simulink model "PMSM_FOC"  (R2022b)
settings: Solver=VariableStepAuto  StartTime=0.0  StopTime=10  MaxStep=1e-6  RelTol=1e-3
values from neighbouring files (symbols this model uses):
  Bm = 0    [PMSM_FOC_parameters.m]
  downlimit_iq = -Vdc/sqrt(3)    [PMSM_FOC_parameters.m]
  downlimit_w = -1.2*Tn    (= -0.357696)    [PMSM_FOC_parameters.m]
  dt = Ts    (= 5e-05)    [PMSM_FOC_parameters.m]
  F = 0.0001    [PMSM_FOC_parameters.m]
  fwb = 50    [PMSM_FOC_parameters.m]
  In = 9.2    [PMSM_FOC_parameters.m]
  J = 0.21e-4    (= 2.1e-05)    [PMSM_FOC_parameters.m]
  ki_iq = Rs*wc    (= 879.645943005)    [PMSM_FOC_parameters.m]
  ki_w = kp_w*wsc/5    (= 1.33977738742)    [PMSM_FOC_parameters.m]
  kp_iq = Lq*wc    (= 0.753982236862)    [PMSM_FOC_parameters.m]
  kp_w = J*wsc/K    (= 0.0213232193851)    [PMSM_FOC_parameters.m]
  ks_iq = 1.5*kp_iq    (= 1.13097335529)    [PMSM_FOC_parameters.m]
  ks_w = 1.5*kp_w    (= 0.0319848290776)    [PMSM_FOC_parameters.m]
  Ld = 0.12e-3    (= 0.00012)    [PMSM_FOC_parameters.m]
  Lq = 0.12e-3    (= 0.00012)    [PMSM_FOC_parameters.m]
  Ls = Ld    (= 0.00012)    [PMSM_FOC_parameters.m]
  n = 3000    [PMSM_FOC_parameters.m]
  p = 4    [PMSM_FOC_parameters.m]
  phis = 0.0054    [PMSM_FOC_parameters.m]
  Rs = 0.14    [PMSM_FOC_parameters.m]
  Tn = 1.5*p*phis*In    (= 0.29808)    [PMSM_FOC_parameters.m]
  Ts = 1/fc    (= 5e-05)    [PMSM_FOC_parameters.m]
  uplimit_iq = Vdc/sqrt(3)    [PMSM_FOC_parameters.m]
  uplimit_w = 1.2*Tn    (= 0.357696)    [PMSM_FOC_parameters.m]
  Vdc = 24    [PMSM_FOC_parameters.m]
undefined symbols (not defined in the file or in its folder): DiscIntNeverNeededParam
libraries: dspsrcs4 x2, spsACVoltageSourceLib x1, spsAlphaBetaZerotodq0Lib x1, simulink x1, spsDCVoltageSourceLib x1, spsPermanentMagnetSynchronousMachineLib x1, spsThreePhaseVIMeasurementLib x1, spsUniversalBridgeLib x1, spsVoltageMeasurementLib x1, spsabctoAlphaBetaZeroLib x1, spsdq0toAlphaBetaZeroLib x1, spspowerguiLib x1
settings Model: Creator=OptiPlex 7090  LastModifiedBy=OptiPlex 7090
settings DebuggingCC: AlgebraicLoopMsg=none  UnconnectedInputMsg=warning  UnconnectedOutputMsg=warning  UnconnectedLineMsg=warning  SFMachineParentedDataDiag=warning
settings ModelReferenceCC: EnableRefExpFcnMdlSchedulingChecks=on
settings RTWCC: DLArmComputeVersion=19.05

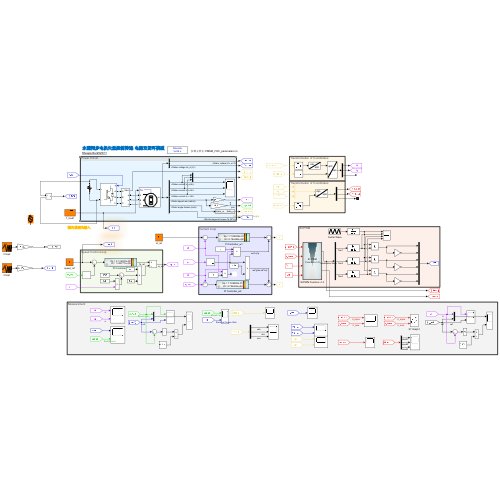
[thumbnail: Simulink's stored preview of the top-level diagram]
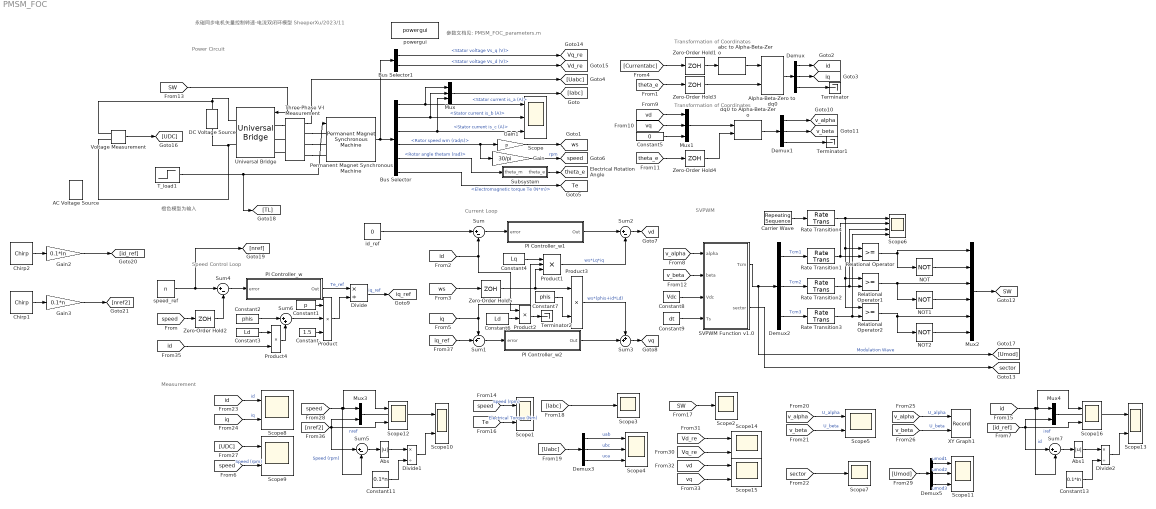
== system PMSM_FOC ==
  note: 参数文档见: PMSM_FOC_parameters.m
  note: Measurement
  note: SVPWM
  note: Speed Control Loop
  note: 橙色模型为输入
  note: Current Loop
  note: Transformation of Coordinates
  note: Power Circuit
  note: 永磁同步电机矢量控制转速-电流双闭环模型
      | SheeperXu/2023/11
  note: Transformation of Coordinates
  AC Voltage Source : spsACVoltageSourceLib/AC Voltage Source  Amplitude=Vdc*0.1  Phase=0  Frequency=500  SampleTime=0  Measurements=None  BusType=swing  Pref=10e3  Qref=0  Qmin=-inf  Qmax=+inf
  Abs : Abs  SaturateOnIntegerOverflow=off
  Abs1 : Abs  SaturateOnIntegerOverflow=off
  Alpha-Beta-Zero to dq0 : spsAlphaBetaZerotodq0Lib/Alpha-Beta-Zero to dq0  Alignment=Aligned with phase A axis
  Bus Selector : BusSelector  OutputSignals=Stator current is_a (A),Stator current is_b (A),Stator current is_c (A),Rotor speed wm (rad/s),Rotor angle thetam (rad),Electromagnetic torque Te (N*m)
  Bus Selector1 : BusSelector  OutputSignals=Stator voltage Vs_q (V),Stator voltage Vs_d (V)
  Carrier Wave : simulink/Sources/Repeating Sequence  rep_seq_t=[0 Ts/2 Ts]  rep_seq_y=[0 Ts/2 0]
  Chirp1 : dspsrcs4/Chirp  sweep=Linear  mode=Unidirectional  f0=0  f1=500  t1=10  Tsweep=10  phase=0  Ts=dt  spf=1  datatype=Double  OutputFrames=off
  Chirp2 : dspsrcs4/Chirp  sweep=Linear  mode=Unidirectional  f0=0  f1=5000  t1=10  Tsweep=10  phase=0  Ts=dt  spf=1  datatype=Double  OutputFrames=off
  Constant : Constant  Value=1.5
  Constant1 : Constant  Value=p
  Constant11 : Constant  Value=0.1*n
  Constant13 : Constant  Value=0.1*In
  Constant2 : Constant  Value=phis
  Constant3 : Constant  Value=Ld
  Constant4 : Constant  Value=Lq
  Constant5 : Constant  Value=0
  Constant6 : Constant  Value=Ld
  Constant7 : Constant  Value=phis
  Constant8 : Constant  Value=Vdc
  Constant9 : Constant  Value=dt
  DC Voltage Source : spsDCVoltageSourceLib/DC Voltage Source  Amplitude=Vdc  Measurements=None
  Demux{,1..3,5} (5 alike) : Demux  Outputs=3
  Divide : Product  Inputs=*/
  Divide1 : Product  Inputs=*/
  Divide2 : Product  Inputs=*/
  Gain : Gain  Gain=30/pi
  Gain1 : Gain  Gain=p
  Gain2 : Gain  Gain=0.1*In
  Gain3 : Gain  Gain=0.1*n
  Mux : Mux  Inputs=3
  Mux1 : Mux  Inputs=3
  Mux2 : Mux  Inputs=6
  Mux3 : Mux  Inputs=2
  Mux4 : Mux  Inputs=2
  NOT : Logic  Operator=NOT  IconShape=distinctive  AllPortsSameDT=off  OutDataTypeStr=boolean
  NOT1 : Logic  Operator=NOT  IconShape=distinctive  AllPortsSameDT=off  OutDataTypeStr=boolean
  NOT2 : Logic  Operator=NOT  IconShape=distinctive  AllPortsSameDT=off  OutDataTypeStr=boolean
  PI Controller_w : Subsystem  mask{Kp=kp_w, Ki=ki_w, Ks=ks_w, uplimit=uplimit_w, downlimit=downlimit_w, SampleTime=1/fwb}
      mask prompts: uplimit "Up_Limit"; downlimit "Down_Limit"; SampleTime "Sample_Time(s)"
      mask DialogControl DescTextVar Prompt: PI Controller
      mask DialogControl ParameterGroupVar Prompt: 参数
      mask DialogControl Control2 Prompt: PI Controller Parameters
      mask Display:
      | image('PI.png');
      | fprintf('Kp = %d\n Ki= %d', Kp, Ki);
  PI Controller_w1 : Subsystem  mask{Kp=kp_iq, Ki=ki_iq, Ks=ks_iq, uplimit=uplimit_iq, downlimit=downlimit_iq, SampleTime=dt}
      mask prompts: uplimit "Up_Limit"; downlimit "Down_Limit"; SampleTime "Sample_Time(s)"
      mask DialogControl DescTextVar Prompt: PI Controller
      mask DialogControl ParameterGroupVar Prompt: 参数
      mask DialogControl Control2 Prompt: PI Controller Parameters
      mask Display:
      | image('PI.png');
      | fprintf('Kp = %d\n Ki= %d', Kp, Ki);
  PI Controller_w2 : Subsystem  mask{Kp=kp_iq, Ki=ki_iq, Ks=ks_iq, uplimit=uplimit_iq, downlimit=downlimit_iq, SampleTime=dt}
      mask prompts: uplimit "Up_Limit"; downlimit "Down_Limit"; SampleTime "Sample_Time(s)"
      mask DialogControl DescTextVar Prompt: PI Controller
      mask DialogControl ParameterGroupVar Prompt: 参数
      mask DialogControl Control2 Prompt: PI Controller Parameters
      mask Display:
      | image('PI.png');
      | fprintf('Kp = %d\n Ki= %d', Kp, Ki);
  Permanent Magnet Synchronous Machine : spsPermanentMagnetSynchronousMachineLib/Permanent Magnet Synchronous Machine  NbPhases=3  FluxDistribution=Sinusoidal  RotorType=Salient-pole  MechanicalLoad=Torque Tm  PresetModel=No  ShowDetailedParameters=on  MeasurementBus=off  Resistance=Rs  Inductance=8.5e-3  dqInductances=[Ld,Lq]  La=[Ls]  MachineConstant=Flux linkage established by magnets (V.s)  Flux=phis  VoltageCst=3.9178  TorqueCst=0.0324  Flat=120  Mechanical=[J F p 0]  PolePairs=4  InitialConditions=[0,0, 0,0]  InitialConditions5ph=[0 0 0 0 0 0]  RefAngle=Aligned with phase A axis (original Park)  IterativeDiscreteModel=Trapezoidal non iterative  TsBlock=-1  TsPowergui=0
  Product : Product  Inputs=3
  Product1 : Product  Inputs=3
  Product2 : Product
  Product3 : Product
  Product4 : Product
  Rate Transition{1..4} (4 alike) : RateTransition  Deterministic=off
  Relational Operator : RelationalOperator  OutDataTypeStr=boolean  RndMeth=Simplest  InputSameDT=off
  Relational Operator1 : RelationalOperator  OutDataTypeStr=boolean  RndMeth=Simplest  InputSameDT=off
  Relational Operator2 : RelationalOperator  OutDataTypeStr=boolean  RndMeth=Simplest  InputSameDT=off
  SVPWM Function v1.0 : MATLAB Function  TreatAsAtomicUnit=on
  Scope : Scope  NumInputPorts=3
  Scope{1,5,8..10,12..16} (10 alike) : Scope  NumInputPorts=2
  Scope11 : Scope  NumInputPorts=3
  Scope2 : Scope
  Scope3 : Scope
  Scope4 : Scope  NumInputPorts=3
  Scope6 : Scope  NumInputPorts=4
  Scope7 : Scope
  Subsystem : Subsystem
  Sum{,2,4..5,7} (5 alike) : Sum  Inputs=|+-
  Sum1 : Sum  Inputs=-+|
  Sum3 : Sum  Inputs=++|
  Sum6 : Sum  Inputs=|++
  T_load1 : Step  Time=0  Before=0.3*Tn  After=0.3*Tn  SampleTime=dt
  Terminator : Terminator
  Terminator1 : Terminator
  Terminator2 : Terminator
  Three-Phase V-I Measurement : spsThreePhaseVIMeasurementLib/Three-Phase V-I Measurement  VoltageMeasurement=phase-to-phase  SetLabelV=off  LabelV=Vabc  Vpu=off  VpuLL=off  CurrentMeasurement=yes  SetLabelI=on  LabelI=Currentabc  Ipu=off  Pbase=100e6  Vbase=500e3  OutputType=Complex  PhasorSimulation=off  PSBequivalent=0
  Universal Bridge : spsUniversalBridgeLib/Universal Bridge  Arms=3  SnubberResistance=1e5  SnubberCapacitance=inf  Device=IGBT / Diodes  Ron=0.001  Lon=0  ForwardVoltages="[  0  0  ]"  ForwardVoltage=0  GTOparameters=[ 10e-6 , 20e-6 ]  IGBTparameters=[ 1e-6 , 2e-6 ]  Measurements=Device voltages  Measurements_2=None  converterType=Rectifier
  Voltage Measurement : spsVoltageMeasurementLib/Voltage Measurement  PhasorSimulation=off  OutputType=Complex  PSBequivalent=0
  XY Graph1 : Record  FileSettingsInternal="{\"entries\":[{\"content\":{\"excelSettings\":{\"content\":{},\"type\":\"Streamout.ExcelSettings\"}},\"type\":\"Streamout.FileSettingStorage\",\"uuid\":\"a06b98c5-8dbe-469b-b57c-4ceb2281ba3f\"}],\"packageUris\":[\"http://schema.mathworks.com/mf0/streamout_blocks/R2020a\"],\"version\":\"1.0\"}"  Layout=[1 1]  SignalsInternal="{\"entries\":[{\"content\":{\"signals\":[{\"content\":{\"blockPath\":[\"PMSM_FOC/XY Graph1\"],\"channel\":[],\"dimensions\":[1],\"domain\":\"PMSM_FOC/XY Graph1\",\"lineColor\":\"#a2142f\",\"plots\":[1],\"port\":1,\"sid\":[],\"signalID\":17,\"signalName\":\"U_alpha\"},\"type\":\"RecordBlkView.Signal\",\"uuid\":\"add1d3f9-caf3-41c6-8cfa-02cf336879b9\"},{\"content\":{\"blockPath\":[\"PMSM_FOC/XY Graph1\"],\"channel\":[],\"dimensions\":[1],\"domain\":\"PMSM_FOC/XY Graph1\",\"lineColor\":\"#139fff\",\"plots\":[1],\"port\":2,\"sid\":[],\"signalID\":20,\"signalName\":\"U_beta\"},\"type\":\"RecordBlkView.Signal\",\"uuid\":\"8e1dd278-356f-4010-8d5d-71b90ce6082a\"}]},\"type\":\"RecordBlkView.InputSignals\",\"uuid\":\"6cc1d440-9683-4637-b98a-52bf58c64516\"}],\"packageUris\":[\"http://schema.mathworks.com/mf0/streamout_blocks/R2020a\"],\"version\":\"1.0\"}"  VisualizationBindings="{\"xyplotplugin\":{\"info\":[{\"series\":[{\"bindingParametersList\":[{\"parameter\":\"X-Axis\",\"signalID\":17,\"signalName\":\"U_alpha\"},{\"parameter\":\"Y-Axis\",\"signalID\":20,\"signalName\":\"U_beta\"}],\"seriesID\":6900}],\"subplotID\":1}]}}"  CompatibilityTag=XY  st=-1
  Zero-Order Hold{1..5} (5 alike) : ZeroOrderHold  SampleTime=dt
  abc to Alpha-Beta-Zero : spsabctoAlphaBetaZeroLib/abc to Alpha-Beta-Zero
  dq0 to Alpha-Beta-Zero : spsdq0toAlphaBetaZeroLib/dq0 to Alpha-Beta-Zero  Alignment=Aligned with phase A axis
  id_ref : Constant  Value=0
  powergui : spspowerguiLib/powergui  Priority=1  SimulationMode=Discrete  SampleTime=1e-6  frequency=60  Iterations=50  frequencyindice=0  Pbase=100e6  ErrMax=1e-4  UnitsV=kV  UnitsW=MW  buscounter=0  FunctionMessages=off  echomessages=off  EnableUseOfTLC=off  CurrentSourceSwitches=off  DisableSnubberDevices=off  DisableRonSwitches=off  DisableVfSwitches=off  DisplayEquations=off  AutomaticDiscreteSolvers=off  SolverType=Tustin/Backward Euler (TBE)  Interpol=off  ExternalGateDelay=off  methode=off  Ts=100  x0status=blocks  SPID=on  SwTol=0  HookPort=off  NonlinearTolerance=1e-4  nMaxIteration=100  ContinueOnMaxIteration=off  RestoreLinks=warning  ResistiveCurrentMeasurement=off  Frange=[0:2:500]  Ylog=off  Xlog=on  ShowGrid=off  save=off  variable=ZData  structure=0  ZoomFFT=off  StartTime=0.0  cycles=1  DisplayStyle=1  fundamental=60  FreqAxis=off  MaxFrequency=1000  frequencyindicesteady=1  RmsSteady=1  display=off
  speed_ref : Constant  Value=n
  tag scope: SW=global, Te=global, Vd_re=global, Vq_re=global, id=global, iq=global, iq_ref=global, sector=global, speed=global, theta_e=global, v_alpha=global, v_beta=global, vd=global, vq=global, ws=global
  wires:
  Permanent Magnet Synchronous Machine/1 -> Bus Selector/1, Bus Selector1/1
  Bus Selector/2 -> Mux/2, Scope/2  "<Stator current is_b (A)>"
  Bus Selector/1 -> Scope/1, Mux/1  "<Stator current is_a (A)>"
  Bus Selector/3 -> Scope/3, Mux/3  "<Stator current is_c (A)>"
  Bus Selector/4 -> Gain/1, Gain1/1  "<Rotor speed wm (rad/s)>"
  Mux/1 -> [Iabc]
  [Currentabc] -> Zero-Order Hold1/1
  abc to Alpha-Beta-Zero/1 -> Alpha-Beta-Zero to dq0/1
  Alpha-Beta-Zero to dq0/1 -> Demux/1
  Demux/1 -> [id]
  Demux/2 -> [iq]
  Gain2/1 -> [id_ref]
  T_load1/1 -> [TL], Permanent Magnet Synchronous Machine/1
  Sum/1 -> PI Controller_w1/1(error)
  PI Controller_w1/1(Out) -> Sum2/1
  Sum1/1 -> PI Controller_w2/1(error)
  Sum4/1 -> PI Controller_w/1(error)
  Bus Selector/5 -> Subsystem/1(theta_m)  "<Rotor angle thetam (rad)>"
  [speed] -> Zero-Order Hold2/1
  Zero-Order Hold1/1 -> abc to Alpha-Beta-Zero/1
  [theta_e] -> Zero-Order Hold3/1
  Subsystem/1(theta_e) -> [theta_e]
  Gain/1 -> [speed]  "rpm"
  Bus Selector/6 -> [Te]  "<Electromagnetic torque Te (N*m)>"
  Zero-Order Hold2/1 -> Sum4/2
  Zero-Order Hold3/1 -> Alpha-Beta-Zero to dq0/2
  PI Controller_w/1(Out) -> Divide/1  "Te_ref"
  Constant1/1 -> Product/1
  Product/1 -> Divide/2
  Gain1/1 -> [ws]
  Constant4/1 -> Product1/1
  [ws] -> Zero-Order Hold5/1
  PI Controller_w2/1(Out) -> Sum3/2
  [iq] -> Product1/2, Sum1/1
  [id] -> Sum/2, Product2/1
  Constant6/1 -> Product2/2
  Zero-Order Hold5/1 -> Product3/1, Product1/3
  Product1/1 -> Sum2/2  "ws*Lq*iq"
  Product3/1 -> Sum3/1  "ws*(phis+id*Ld)"
  Constant2/1 -> Sum6/1
  Sum6/1 -> Product/2
  Constant3/1 -> Product4/1
  Product4/1 -> Sum6/2
  Constant/1 -> Product/3
  Sum2/1 -> [vd]
  Sum3/1 -> [vq]
  Divide/1 -> [iq_ref]  "iq_ref"
  Mux1/1 -> dq0 to Alpha-Beta-Zero/1
  [vd] -> Mux1/1
  [vq] -> Mux1/2
  Constant5/1 -> Mux1/3
  [theta_e] -> Zero-Order Hold4/1
  Zero-Order Hold4/1 -> dq0 to Alpha-Beta-Zero/2
  dq0 to Alpha-Beta-Zero/1 -> Demux1/1
  Demux1/1 -> [v_alpha]
  Demux1/2 -> [v_beta]
  [v_alpha] -> SVPWM Function v1.0/1(alpha)
  [v_beta] -> SVPWM Function v1.0/2(beta)
  [SW] -> Universal Bridge/1
  Constant8/1 -> SVPWM Function v1.0/3(Vdc)
  Constant9/1 -> SVPWM Function v1.0/4(Ts)
  [speed] -> Scope1/1  "Speed (rpm)"
  Demux/3 -> Terminator/1
  Demux1/3 -> Terminator1/1
  [SW] -> Scope2/1
  [Iabc] -> Scope3/1
  [v_alpha] -> Scope5/1  "U_alpha"
  [v_beta] -> Scope5/2  "U_beta"
  Demux2/1 -> Rate Transition1/1  "Tcm1"
  Demux2/2 -> Rate Transition2/1  "Tcm2"
  Demux2/3 -> Rate Transition3/1  "Tcm3"
  Relational Operator/1 -> Mux2/1, NOT/1
  Relational Operator1/1 -> NOT1/1, Mux2/3
  Relational Operator2/1 -> Mux2/5, NOT2/1
  Mux2/1 -> [SW]
  SVPWM Function v1.0/1(Tcm) -> Demux2/1, [Umod]  "Modulation Wave"
  SVPWM Function v1.0/2(sector) -> [sector]
  [sector] -> Scope7/1
  [id] -> Scope8/1  "id"
  [iq] -> Scope8/2  "iq"
  [Uabc] -> Demux3/1
  Demux3/1 -> Scope4/1  "uab"
  [v_alpha] -> XY Graph1/1  "U_alpha"
  [v_beta] -> XY Graph1/2  "U_beta"
  Demux3/2 -> Scope4/2  "ubc"
  Demux3/3 -> Scope4/3  "uca"
  Three-Phase V-I Measurement/1 -> [Uabc]
  Carrier Wave/1 -> Rate Transition4/1
  Rate Transition1/1 -> Scope6/2, Relational Operator/2
  Rate Transition2/1 -> Scope6/3, Relational Operator1/2
  Rate Transition3/1 -> Scope6/4, Relational Operator2/2
  [Umod] -> Demux5/1
  Demux5/2 -> Scope11/2  "umod2"
  Demux5/1 -> Scope11/1  "umod1"
  Demux5/3 -> Scope11/3  "umod3"
  Bus Selector1/1 -> [Vq_re]  "<Stator voltage Vs_q (V)>"
  Bus Selector1/2 -> [Vd_re]  "<Stator voltage Vs_d (V)>"
  [Vd_re] -> Scope14/1
  [Vq_re] -> Scope14/2
  [vd] -> Scope15/1
  [vq] -> Scope15/2
  [id] -> Product4/2
  Rate Transition4/1 -> Relational Operator2/1, Relational Operator1/1, Relational Operator/1, Scope6/1
  Constant7/1 -> Product3/2
  Product2/1 -> Terminator2/1
  Voltage Measurement/1 -> [UDC]
  [UDC] -> Scope9/1
  [speed] -> Scope9/2  "Speed (rpm)"
  [speed] -> Sum5/2, Scope12/1, Mux3/1  "Speed (rpm)"
  [nref2] -> Scope12/2, Mux3/2, Sum5/1  "nref"
  [Te] -> Scope1/2  "Electrical Torque (Nm)"
  speed_ref/1 -> [nref], Sum4/1
  Mux3/1 -> Scope10/1
  Sum5/1 -> Abs/1
  NOT/1 -> Mux2/2
  NOT1/1 -> Mux2/4
  NOT2/1 -> Mux2/6
  Abs/1 -> Divide1/1
  Constant11/1 -> Divide1/2
  Divide1/1 -> Scope10/2
  Chirp1/1 -> Gain3/1
  Abs1/1 -> Divide2/1
  Constant13/1 -> Divide2/2
  Divide2/1 -> Scope13/2
  [id_ref] -> Scope16/2, Mux4/2, Sum7/1  "iref"
  [id] -> Sum7/2, Scope16/1, Mux4/1  "id"
  Mux4/1 -> Scope13/1
  Sum7/1 -> Abs1/1
  Chirp2/1 -> Gain2/1
  id_ref/1 -> Sum/1
  [iq_ref] -> Sum1/2
  Gain3/1 -> [nref2]
  connections:
  DC Voltage Source/RConn1 -- Voltage Measurement/LConn1 -- Universal Bridge/RConn1
  Universal Bridge/LConn1 -- Three-Phase V-I Measurement/LConn1
  Three-Phase V-I Measurement/LConn2 -- Universal Bridge/LConn2
  Three-Phase V-I Measurement/LConn3 -- Universal Bridge/LConn3
  Three-Phase V-I Measurement/RConn1 -- Permanent Magnet Synchronous Machine/LConn1
  Three-Phase V-I Measurement/RConn2 -- Permanent Magnet Synchronous Machine/LConn2
  Three-Phase V-I Measurement/RConn3 -- Permanent Magnet Synchronous Machine/LConn3
  Voltage Measurement/LConn2 -- DC Voltage Source/LConn1 -- Universal Bridge/RConn2

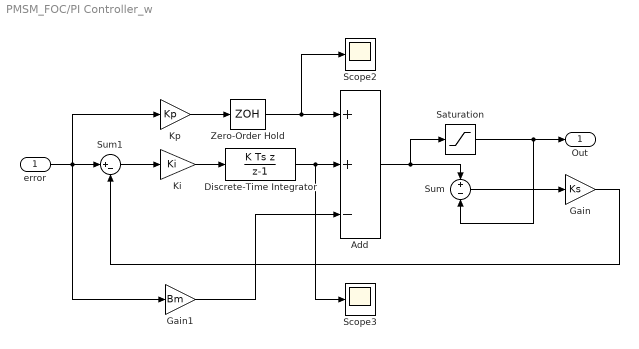
== system PMSM_FOC/PI Controller_w ==
  error : Inport
  Add : Sum  Inputs=++-
  Discrete-Time Integrator : DiscreteIntegrator  IntegratorMethod=Integration: Backward Euler  SampleTime=dt  LimitOutput=on  UpperSaturationLimit=uplimit  LowerSaturationLimit=downlimit  ICPrevOutput=DiscIntNeverNeededParam  ICPrevScaledInput=DiscIntNeverNeededParam
  Gain : Gain  Gain=Ks
  Gain1 : Gain  Gain=Bm
  Ki : Gain  Gain=Ki
  Kp : Gain  Gain=Kp
  Saturation : Saturate  UpperLimit=uplimit  LowerLimit=downlimit
  Scope2 : Scope
  Scope3 : Scope
  Sum : Sum  Inputs=+|-
  Sum1 : Sum  Inputs=|+-
  Zero-Order Hold : ZeroOrderHold  SampleTime=dt
  Out : Outport
  wires:
  Kp/1 -> Zero-Order Hold/1
  error/1 -> Gain1/1, Sum1/1, Kp/1
  Zero-Order Hold/1 -> Scope2/1, Add/1
  Add/1 -> Saturation/1, Sum/1
  Saturation/1 -> Sum/2, Out/1
  Sum/1 -> Gain/1
  Gain/1 -> Sum1/2
  Sum1/1 -> Ki/1
  Ki/1 -> Discrete-Time Integrator/1
  Discrete-Time Integrator/1 -> Scope3/1, Add/2
  Gain1/1 -> Add/3

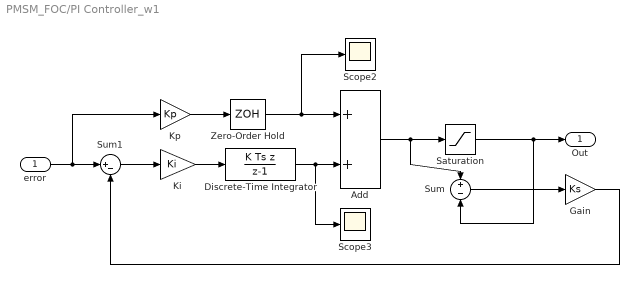
== system PMSM_FOC/PI Controller_w1 ==
  error : Inport
  Add : Sum
  Discrete-Time Integrator : DiscreteIntegrator  IntegratorMethod=Integration: Backward Euler  SampleTime=dt  LimitOutput=on  UpperSaturationLimit=uplimit  LowerSaturationLimit=downlimit  ICPrevOutput=DiscIntNeverNeededParam  ICPrevScaledInput=DiscIntNeverNeededParam
  Gain : Gain  Gain=Ks
  Ki : Gain  Gain=Ki
  Kp : Gain  Gain=Kp
  Saturation : Saturate  UpperLimit=uplimit  LowerLimit=downlimit
  Scope2 : Scope
  Scope3 : Scope
  Sum : Sum  Inputs=+|-
  Sum1 : Sum  Inputs=|+-
  Zero-Order Hold : ZeroOrderHold  SampleTime=dt
  Out : Outport
  wires:
  Discrete-Time Integrator/1 -> Add/2, Scope3/1
  Ki/1 -> Discrete-Time Integrator/1
  Sum1/1 -> Ki/1
  Gain/1 -> Sum1/2
  Sum/1 -> Gain/1
  Saturation/1 -> Out/1, Sum/2
  Add/1 -> Saturation/1, Sum/1
  Zero-Order Hold/1 -> Scope2/1, Add/1
  error/1 -> Kp/1, Sum1/1
  Kp/1 -> Zero-Order Hold/1

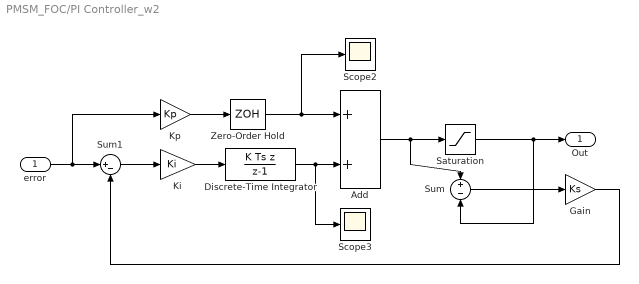
== system PMSM_FOC/PI Controller_w2 ==
  error : Inport
  Add : Sum
  Discrete-Time Integrator : DiscreteIntegrator  IntegratorMethod=Integration: Backward Euler  SampleTime=dt  LimitOutput=on  UpperSaturationLimit=uplimit  LowerSaturationLimit=downlimit  ICPrevOutput=DiscIntNeverNeededParam  ICPrevScaledInput=DiscIntNeverNeededParam
  Gain : Gain  Gain=Ks
  Ki : Gain  Gain=Ki
  Kp : Gain  Gain=Kp
  Saturation : Saturate  UpperLimit=uplimit  LowerLimit=downlimit
  Scope2 : Scope
  Scope3 : Scope
  Sum : Sum  Inputs=+|-
  Sum1 : Sum  Inputs=|+-
  Zero-Order Hold : ZeroOrderHold  SampleTime=dt
  Out : Outport
  wires:
  Kp/1 -> Zero-Order Hold/1
  error/1 -> Sum1/1, Kp/1
  Zero-Order Hold/1 -> Add/1, Scope2/1
  Add/1 -> Sum/1, Saturation/1
  Saturation/1 -> Sum/2, Out/1
  Sum/1 -> Gain/1
  Gain/1 -> Sum1/2
  Sum1/1 -> Ki/1
  Ki/1 -> Discrete-Time Integrator/1
  Discrete-Time Integrator/1 -> Scope3/1, Add/2

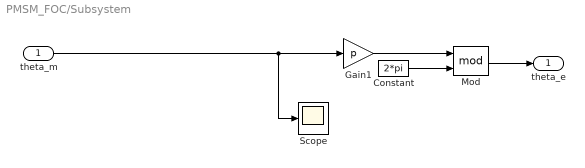
== system PMSM_FOC/Subsystem ==
  theta_m : Inport
  Constant : Constant  Value=2*pi
  Gain1 : Gain  Gain=p
  Mod : Math  Operator=mod
  Scope : Scope
  theta_e : Outport
  wires:
  Constant/1 -> Mod/2
  Mod/1 -> theta_e/1
  Gain1/1 -> Mod/1
  theta_m/1 -> Scope/1, Gain1/1

== matlab function PMSM_FOC/SVPWM Function v1.0 ==
  data: alpha input; beta input; Vdc input; Ts input; Tcm output; sector output
%------------------------------------------------------------
%   SVPWM Function  v1.0
%   Editor: Sheeper Xu
%   Data: 2023/11
%------------------------------------------------------------
function [Tcm,sector] = fcn(alpha, beta, Vdc, Ts)
%输出变量初始化
    tcm1=0;
    tcm2=0;
    tcm3=0;
%判断中间变量
    ref1=beta;
    ref2=-1/2*beta+sqrt(3)*alpha/2;
    ref3=-1/2*beta-sqrt(3)*alpha/2;
%扇区判断
    if(ref1>0)        
        a=1;
    else        
        a=0;
    end
    if(ref2>0)         
        b=1;
    else         
        b=0;
    end
    if(ref3>0)       
        c=1;
    else        
        c=0;
    end
    sector=4*c+2*b+a; %扇区选择数计算
%------------------------------------------------------------
    % 扇区-sector 映射
    %扇区      I  II  III  IV  V  VI
    % sector 3  1  5   4   6  12
%------------------------------------------------------------
%设置矢量作用时间中间量
    X=Ts*sqrt(3)/Vdc*beta;
    Y=Ts*sqrt(3)/Vdc*(sqrt(3)*alpha+beta)/2;
    Z=Ts*sqrt(3)/Vdc*(-sqrt(3)*alpha+beta)/2;
%------------------------------------------------------------
% sector-矢量作用时间中间量映射
    % sector   1    2    3    4   5    6  
    %    t1       Z   Y   -Z  -X   X   -Y
    %    t2       Y  -X    X   Z  -Y   -Z
    %    t0            Ts-t1-t2
%------------------------------------------------------------
% 矢量作用时间计算
 switch(sector)
        case 1
            t1=Z;            
            t2=Y;
        case 2
            t1=Y;           
            t2=-X;
        case 3
            t1=-Z;           
            t2=X;
        case 4
            t1=-X;       
            t2=Z;
        case 5
            t1=X;       
            t2=-Y;
     otherwise
            t1=-Y;       
            t2=-Z;
 end
%过调制处理
if((t1+t2)>Ts)
    t1=Ts*(t1/(t1+t2));
    t2=Ts*(t2/(t1+t2));
end
 t0=(Ts-t1-t2)/2; %零矢量作用时间

%开关切换时间计算(7段式）
    %设置中间变量ta,tb,tc
    ta=t0/2; 
    tb=ta+t1/2; 
    tc=tb+t2/2; 
    %设置a,b,c开关的切换时间分别为tcm1,tcm2,tmc3
%------------------------------------------------------------
    % sector-开关切换时间映射关系
    %   N     1   2   3   4   5   6
    % tcm1 tb  ta  ta  tc  tc  tb
    % tcm2 ta  tc  tb  tb  ta  tc
    % tcm3 tc  tb  tc  ta  tb  ta
%------------------------------------------------------------
switch(sector)
    case 1
        tcm1=tb;    tcm2=ta;    tcm3=tc;
    case 2
        tcm1=ta;    tcm2=tc;    tcm3=tb;
    case 3
        tcm1=ta;    tcm2=tb;    tcm3=tc;
    case 4
        tcm1=tc;    tcm2=tb;    tcm3=ta;
    case 5
        tcm1=tc;    tcm2=ta;    tcm3=tb;
    case 6
        tcm1=tb;    tcm2=tc;    tcm3=ta;
end 

Tcm=[tcm1,tcm2,tcm3]; %输出开关切换时间
